simulink model "furuta_block_model_fixed"  (R2026b)
settings: Solver=FixedStepDiscrete  StopTime=5  FixedStep=.005  EnableMultiTasking=on
InitFcn:
  | validate_furuta_fixed_test('furuta_block_model_fixed');
model workspace (MAT data in the model file):
  calibration = [73.65 -1 4058.5 1]
  controlPeriod = 0.01
  drive = [-1 1.5 1.5 inf]
  driveElectrical : object (value not decoded)
  failureReplayEnabled = 0
  failureReplaySlowdown = 10
  failureReplaySource = 'C:\Capstone1\matlab_furuta\results\ppo_rmd_candidate_tpa79dc374_f9fe_4d66_a12a_2e210f4a8415\ppo_start_-20_+20_armrate_20_current_1.5_time_10_armlimit_Inf.mat'
  failureReplayStartDeg = 20
  failureReplayState = [0 0.1 0.2 0.3 0.4 0.5 0.6 0.7 0.8 0.9 1 1.1 ... (205 elements, 41x5)]
  furutaPPOAgent : rl.agent.rlPPOAgent (value not decoded)
  furutaSACAgent : rl.agent.rlSACAgent (value not decoded)
  furutaToolboxMpc : object (value not decoded)
  initialState = [0; 3.05432619099; 0; 0]
  integrationStep = 0.002
  limits = [inf 3.3 15 20]
  lqrGain = [-1.90684760658 -25.0276005412 -1.03983138576 -2.50199272238]
  maxTorque = 3.15
  milVelocityLimits = [15 25]
  pidGains = [25.0276005412 5.00398544475 1.90684760658 2.07966277151 0.001]
  plantCoefficients = [0.05 0.00016078 0.00016134 0.00013805 0.016934 0.0001 1e-05 0.63]
  rlRewardLevel = 2
  rmd : object (value not decoded)
  rmdCommandDelaySamples = 1
  scenarioStimulus = [0  0  0  0; 20  0  0  0]
  swingLqrThresholds = [0.226892802759 0.2 0.523598775598]
  usePolicyCallback = 0
  useRmd = 1
  velocityFilterTau = 0.03
values from neighbouring files (symbols this model uses):
  C = [B A*B A^2*B A^3*B]    [build_furuta_rmd.m]
  N = 20    [build_furuta_rl.m]    (also in design_classical.m)
  s = load(matFile,'ds')    [analyze_pi_current_run.m]    (also in analyze_pi_speed_run.m; build_furuta_rl.m = sin(x(2));"; build_furuta_simulink.m = s(1); design_classical.m = furuta_scenarios)
  source = [step '/1']    [add_furuta_plant_blocks.m]    (also in build_furuta_pi.m = get_param(line,'SrcPortHandle'); build_furuta_pi_hardware.m = 'Drive interlocks/3'; compare_furuta_actuators.m = get_param([harness '/Requested torque'],'PortHandles'))
  Z = expm([A B; zeros(1,5)]*p.Ts)    [furuta_linearize.m]
symbols that are objects in the model workspace (value not decoded): driveElectrical, rmd
undefined symbols (not defined in the file or in its folder): lmpcF, lmpcH, poleGain, sgn, X, Y
libraries: sm_lib x36, raspberrypiCommlib x9, nesl_utility x8, fl_lib x7, rllib x2, mpclib x1, slpidlib x1, ee_lib x1
(part 2 of 4)

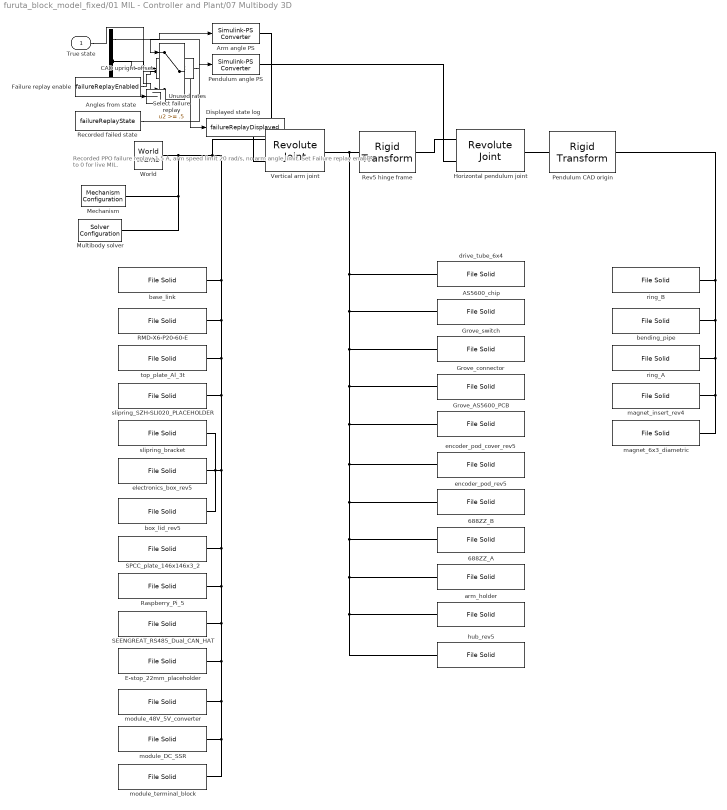
== system furuta_block_model_fixed/01 MIL - Controller and Plant/07 Multibody 3D ==
  note: Recorded PPO failure replay: 1.5 A, arm speed limit 20 rad/s, no arm angle limit. Set Failure replay enable to 0 for live MIL.
  True state : Inport
  688ZZ_A : sm_lib/Body Elements/File Solid  ExtGeomFileName=C:/Capstone1/models/rev5/source/meshes/688ZZ_A.stl  UnitType=Custom  ExtGeomFileUnits=mm  StepReaderType=HEX  ExportConvexHullGeometry=off  InertiaType=Custom  BasedOnType=DensityFromFile  Density=1000  DensityUnits=kg/m^3  Mass=0.005918760559363255  MassUnits=kg  CenterOfMass=[0.016 -2.788462968231947e-13 0.018]  CenterOfMassUnits=m  MomentsOfInertia=[2.367504233937143e-07 1.307059618430119e-07 1.307059638813835e-07]  MomentsOfInertiaUnits=kg*m^2  ProductsOfInertia=[7.843725669008149e-23 0 2.614575223002716e-23]  ProductsOfInertiaUnits=kg*m^2  GraphicType=FromGeometry  MarkerShape=Sphere  MarkerSize=10  GraphicVisPropType=SimpleVisualProperties  GraphicDiffuseColor=[.20 .50 .78]  GraphicOpacity=1  GraphicSpecularColor=[0.5 0.5 0.5 1.0]  GraphicAmbientColor=[0.15 0.15 0.15 1.0]  GraphicEmissiveColor=[0.0 0.0 0.0 1.0]  GraphicShininess=75  DoExposeReferenceFrame=on  SerializedFrames=<Frames/>
  688ZZ_B : sm_lib/Body Elements/File Solid  ExtGeomFileName=C:/Capstone1/models/rev5/source/meshes/688ZZ_B.stl  UnitType=Custom  ExtGeomFileUnits=mm  StepReaderType=HEX  ExportConvexHullGeometry=off  InertiaType=Custom  BasedOnType=DensityFromFile  Density=1000  DensityUnits=kg/m^3  Mass=0.005918760559363255  MassUnits=kg  CenterOfMass=[-0.016 -2.788462968231947e-13 0.018]  CenterOfMassUnits=m  MomentsOfInertia=[2.367504233937143e-07 1.307059618430119e-07 1.307059638813835e-07]  MomentsOfInertiaUnits=kg*m^2  ProductsOfInertia=[7.843725669008149e-23 4.235164736271502e-22 -1.13298259663451e-22]  ProductsOfInertiaUnits=kg*m^2  GraphicType=FromGeometry  MarkerShape=Sphere  MarkerSize=10  GraphicVisPropType=SimpleVisualProperties  GraphicDiffuseColor=[.20 .50 .78]  GraphicOpacity=1  GraphicSpecularColor=[0.5 0.5 0.5 1.0]  GraphicAmbientColor=[0.15 0.15 0.15 1.0]  GraphicEmissiveColor=[0.0 0.0 0.0 1.0]  GraphicShininess=75  DoExposeReferenceFrame=on  SerializedFrames=<Frames/>
  AS5600_chip : sm_lib/Body Elements/File Solid  ExtGeomFileName=C:/Capstone1/models/rev5/source/meshes/AS5600_chip.stl  UnitType=Custom  ExtGeomFileUnits=mm  StepReaderType=HEX  ExportConvexHullGeometry=off  InertiaType=Custom  BasedOnType=DensityFromFile  Density=1000  DensityUnits=kg/m^3  Mass=0.0002354999999999998  MassUnits=kg  CenterOfMass=[-0.02765 0 0.018]  CenterOfMassUnits=m  MomentsOfInertia=[8.04625000000029e-10 3.581562500000463e-10 5.347812500000514e-10]  MomentsOfInertiaUnits=kg*m^2  ProductsOfInertia=[-3.404394821604484e-25 2.646977960169689e-23 1.021318446481345e-24]  ProductsOfInertiaUnits=kg*m^2  GraphicType=FromGeometry  MarkerShape=Sphere  MarkerSize=10  GraphicVisPropType=SimpleVisualProperties  GraphicDiffuseColor=[.20 .50 .78]  GraphicOpacity=1  GraphicSpecularColor=[0.5 0.5 0.5 1.0]  GraphicAmbientColor=[0.15 0.15 0.15 1.0]  GraphicEmissiveColor=[0.0 0.0 0.0 1.0]  GraphicShininess=75  DoExposeReferenceFrame=on  SerializedFrames=<Frames/>
  Angles from state : Demux  Outputs=[1 1 2]
  Arm angle PS : nesl_utility/Simulink-PS Converter  PhysicalDomain=network_engine_domain  SubClassName=ps_input  LeftPortType=input  RightPortType=output  PseudoPeriodic=off  Frequencies=[]  NoiseDistribution=none  NoiseParameters=[]  Unit=rad  AffineConversion=off  FilteringAndDerivatives=filter  SimscapeFilterOrder=2  InputFilterTimeConstant=.003  UdotUserProvided=0
  CAD upright offset : Bias  Bias=-pi/2  SaturateOnIntegerOverflow=off
  Displayed state log : ToWorkspace  VariableName=failureReplayDisplayed  SaveFormat=Timeseries  SampleTime=-1
  E-stop_22mm_placeholder : sm_lib/Body Elements/File Solid  ExtGeomFileName=C:/Capstone1/models/rev5/source/meshes/E-stop_22mm_placeholder.stl  UnitType=Custom  ExtGeomFileUnits=mm  StepReaderType=HEX  ExportConvexHullGeometry=off  InertiaType=Custom  BasedOnType=DensityFromFile  Density=1000  DensityUnits=kg/m^3  Mass=0.1193616712804906  MassUnits=kg  CenterOfMass=[0.04499999999999998 -0.0525 -0.1708]  CenterOfMassUnits=m  MomentsOfInertia=[1.952558006030128e-05 7.221381112470972e-06 1.95255800603003e-05]  MomentsOfInertiaUnits=kg*m^2  ProductsOfInertia=[-8.673617379884035e-19 8.673617379884035e-19 0]  ProductsOfInertiaUnits=kg*m^2  GraphicType=FromGeometry  MarkerShape=Sphere  MarkerSize=10  GraphicVisPropType=SimpleVisualProperties  GraphicDiffuseColor=[.42 .43 .46]  GraphicOpacity=1  GraphicSpecularColor=[0.5 0.5 0.5 1.0]  GraphicAmbientColor=[0.15 0.15 0.15 1.0]  GraphicEmissiveColor=[0.0 0.0 0.0 1.0]  GraphicShininess=75  DoExposeReferenceFrame=on  SerializedFrames=<Frames/>
  Failure replay enable : Constant  Value=failureReplayEnabled
  Grove_AS5600_PCB : sm_lib/Body Elements/File Solid  ExtGeomFileName=C:/Capstone1/models/rev5/source/meshes/Grove_AS5600_PCB.stl  UnitType=Custom  ExtGeomFileUnits=mm  StepReaderType=HEX  ExportConvexHullGeometry=off  InertiaType=Custom  BasedOnType=DensityFromFile  Density=1000  DensityUnits=kg/m^3  Mass=0.0023511221076278556  MassUnits=kg  CenterOfMass=[-0.0292 -0.009998882871009487 0.018]  CenterOfMassUnits=m  MomentsOfInertia=[3.903658018417303e-07 7.840966792904181e-08 3.129592793452765e-07]  MomentsOfInertiaUnits=kg*m^2  ProductsOfInertia=[1.058791184067875e-22 2.117582368135751e-22 0]  ProductsOfInertiaUnits=kg*m^2  GraphicType=FromGeometry  MarkerShape=Sphere  MarkerSize=10  GraphicVisPropType=SimpleVisualProperties  GraphicDiffuseColor=[.20 .50 .78]  GraphicOpacity=1  GraphicSpecularColor=[0.5 0.5 0.5 1.0]  GraphicAmbientColor=[0.15 0.15 0.15 1.0]  GraphicEmissiveColor=[0.0 0.0 0.0 1.0]  GraphicShininess=75  DoExposeReferenceFrame=on  SerializedFrames=<Frames/>
  Grove_connector : sm_lib/Body Elements/File Solid  ExtGeomFileName=C:/Capstone1/models/rev5/source/meshes/Grove_connector.stl  UnitType=Custom  ExtGeomFileUnits=mm  StepReaderType=HEX  ExportConvexHullGeometry=off  InertiaType=Custom  BasedOnType=DensityFromFile  Density=1000  DensityUnits=kg/m^3  Mass=0.0005172800000000002  MassUnits=kg  CenterOfMass=[-0.0325 -0.02 0.018]  CenterOfMassUnits=m  MomentsOfInertia=[9.174822933333419e-09 7.493662933333236e-09 3.836493333333296e-09]  MomentsOfInertiaUnits=kg*m^2  ProductsOfInertia=[2.646977960169689e-23 0 0]  ProductsOfInertiaUnits=kg*m^2  GraphicType=FromGeometry  MarkerShape=Sphere  MarkerSize=10  GraphicVisPropType=SimpleVisualProperties  GraphicDiffuseColor=[.20 .50 .78]  GraphicOpacity=1  GraphicSpecularColor=[0.5 0.5 0.5 1.0]  GraphicAmbientColor=[0.15 0.15 0.15 1.0]  GraphicEmissiveColor=[0.0 0.0 0.0 1.0]  GraphicShininess=75  DoExposeReferenceFrame=on  SerializedFrames=<Frames/>
  Grove_switch : sm_lib/Body Elements/File Solid  ExtGeomFileName=C:/Capstone1/models/rev5/source/meshes/Grove_switch.stl  UnitType=Custom  ExtGeomFileUnits=mm  StepReaderType=HEX  ExportConvexHullGeometry=off  InertiaType=Custom  BasedOnType=DensityFromFile  Density=1000  DensityUnits=kg/m^3  Mass=6.268416000000009e-05  MassUnits=kg  CenterOfMass=[-0.0316 -0.0139 0.01292]  CenterOfMassUnits=m  MomentsOfInertia=[2.684971520000019e-10 2.810339839999896e-10 9.444413439999819e-11]  MomentsOfInertiaUnits=kg*m^2  ProductsOfInertia=[0 -3.308722450212111e-24 -3.308722450212111e-24]  ProductsOfInertiaUnits=kg*m^2  GraphicType=FromGeometry  MarkerShape=Sphere  MarkerSize=10  GraphicVisPropType=SimpleVisualProperties  GraphicDiffuseColor=[.20 .50 .78]  GraphicOpacity=1  GraphicSpecularColor=[0.5 0.5 0.5 1.0]  GraphicAmbientColor=[0.15 0.15 0.15 1.0]  GraphicEmissiveColor=[0.0 0.0 0.0 1.0]  GraphicShininess=75  DoExposeReferenceFrame=on  SerializedFrames=<Frames/>
  Horizontal pendulum joint : sm_lib/Joints/Revolute Joint  JointMode=Normal  CompositeWrenchDir=FollowerOnBase  CompositeWrenchFrame=BaseFrame  SenseConstraintForce=off  SenseConstraintTorque=off  SenseTotalForce=off  SenseTotalTorque=off  PositionTargetSpecify=off  PositionTargetPriority=High  PositionTargetValue=0  PositionTargetValueUnits=deg  VelocityTargetSpecify=off  VelocityTargetPriority=High  VelocityTargetValue=0  VelocityTargetValueUnits=deg/s  EquilibriumPosition=0  EquilibriumPositionUnits=deg  SpringStiffness=0  SpringStiffnessUnits=N*m/deg  DampingCoefficient=0  DampingCoefficientUnits=N*m/(deg/s)  LowerLimitSpecify=off  LowerLimitBound=-90  LowerLimitBoundUnits=deg  LowerLimitStiffness=1e4  LowerLimitStiffnessUnits=N*m/deg  LowerLimitDamping=10  LowerLimitDampingUnits=N*m/(deg/s)  LowerLimitTransitionRegionWidth=0.1  LowerLimitTransitionRegionWidthUnits=deg  UpperLimitSpecify=off  UpperLimitBound=90  UpperLimitBoundUnits=deg  UpperLimitStiffness=1e4  UpperLimitStiffnessUnits=N*m/deg  UpperLimitDamping=10  UpperLimitDampingUnits=N*m/(deg/s)  UpperLimitTransitionRegionWidth=0.1  UpperLimitTransitionRegionWidthUnits=deg  TorqueActuationMode=ComputedTorque  MotionActuationMode=InputMotion  SensePosition=off  SenseVelocity=off  SenseAcceleration=off  SenseTorqueForce=off  SenseLowerLimitTorqueForce=off  SenseUpperLimitTorqueForce=off
  Mechanism : sm_lib/Utilities/Mechanism Configuration  UniformGravity=Constant  GravityVector=[0 0 -9.80665]  GravityVectorUnits=m/s^2  LinearizationDelta=0.001  JointModeTransitionNonlinearIterations=2
  Multibody solver : nesl_utility/Solver Configuration  PhysicalDomain=network_engine_domain  SubClassName=solver  LeftPortType=input  RightPortType=generic  Tones=[]  Harmonics=[]  SimulateNoise=off  Profile=off  UseLocalSampling=off  EnableSwitchedLinearOptims=on  FrequencyDomain=off  UseCCode=off  RelTol=0.001  AbsTol=0.001  MinStep=1e-09  ToWorkspace=off  RevertToSquareIcSolve=off  NumHomotopyIterations=100  PhasorMode=off  PhasorModeNumHarmonics=1  ConsistencySolver=NEWTON_XTOL_AFTER_FTOL  CanonicalOrdering=CANONICAL  OptimizeIntermediates=OPTIMIZED  MulticoreSolverChoice=BACKWARD_EULER  IndexReductionMethod=DerivativeReplacement  DoDC=off  ResidualTolerance=1e-09  ConsistencyTolSource=GLOBAL  ConsistencyAbsTol=0.001  ConsistencyRelTol=0.001  ConsistencyTolFactor=0.001  UseLocalSolver=off  LocalSolverChoice=NE_BACKWARD_EULER_ADVANCER  ResolveIndetEquations=on  FunctionEvalNumThread=1  LocalSolverSampleTime=0.001  DoFixedCost=off  MaxNonlinIter=3  MaxModeIter=2  ComputeImpulses=off  ImpulseIterations=2  LinearAlgebra=auto  LinearAlgebraNumThread=0  EquationFormulation=NE_TIME_EF  DelaysMemoryBudget=1024  AutomaticFiltering=on  FilteringTimeConstant=0.001  PartitionStorageMethod=AS_NEEDED  PartitionMemoryBudget=1024  PartitionMethod=BALANCED  MultibodyUseLocalSolver=off  MultibodyLocalSolverChoice=ODE1  MultibodyLocalSolverSampleTime=0.001
  Pendulum CAD origin : sm_lib/Frames and Transforms/Rigid Transform  RotationMethod=RotationMatrix  FollAlignAxisA=+X  BaseAlignAxisA=+Y  FollAlignAxisB=+Y  BaseAlignAxisB=+Z  RotationStandardAxis=+Z  RotationAngle=0  RotationAngleUnits=deg  RotationArbitraryAxis=[0 0 1]  RotationSequenceAxes=FollowerAxes  RotationSequence=XYX  RotationSequenceAngles=[0 0 0]  RotationSequenceAnglesUnits=deg  RotationMatrix=[0 0 -1;0 1 0;1 0 0]  Quaternion=[1 0 0 0]  TranslationMethod=Cartesian  TranslationCartesianOffset=[0.018 0 0.0185]  TranslationCartesianOffsetUnits=m  TranslationStandardAxis=+Z  TranslationStandardOffset=0  TranslationStandardOffsetUnits=m  TranslationROffset=0  TranslationROffsetUnits=m  TranslationThetaOffset=0  TranslationThetaOffsetUnits=deg  TranslationZOffset=0  TranslationZOffsetUnits=m
  Pendulum angle PS : nesl_utility/Simulink-PS Converter  PhysicalDomain=network_engine_domain  SubClassName=ps_input  LeftPortType=input  RightPortType=output  PseudoPeriodic=off  Frequencies=[]  NoiseDistribution=none  NoiseParameters=[]  Unit=rad  AffineConversion=off  FilteringAndDerivatives=filter  SimscapeFilterOrder=2  InputFilterTimeConstant=.003  UdotUserProvided=0
  RMD-X6-P20-60-E : sm_lib/Body Elements/File Solid  ExtGeomFileName=C:/Capstone1/models/rev5/source/meshes/RMD-X6-P20-60-E.stl  UnitType=Custom  ExtGeomFileUnits=mm  StepReaderType=HEX  ExportConvexHullGeometry=off  InertiaType=Custom  BasedOnType=DensityFromFile  Density=1000  DensityUnits=kg/m^3  Mass=0.5295460172821769  MassUnits=kg  CenterOfMass=[-8.898918041415573e-05 -0.0001349554467787079 -0.02861574603154959]  CenterOfMassUnits=m  MomentsOfInertia=[0.0005329118585045489 0.0005318244984692392 0.0005420384995759367]  MomentsOfInertiaUnits=kg*m^2  ProductsOfInertia=[-2.743134480207274e-06 -1.937494531495924e-06 7.067599187778668e-07]  ProductsOfInertiaUnits=kg*m^2  GraphicType=FromGeometry  MarkerShape=Sphere  MarkerSize=10  GraphicVisPropType=SimpleVisualProperties  GraphicDiffuseColor=[.42 .43 .46]  GraphicOpacity=1  GraphicSpecularColor=[0.5 0.5 0.5 1.0]  GraphicAmbientColor=[0.15 0.15 0.15 1.0]  GraphicEmissiveColor=[0.0 0.0 0.0 1.0]  GraphicShininess=75  DoExposeReferenceFrame=on  SerializedFrames=<Frames/>
  Raspberry_Pi_5 : sm_lib/Body Elements/File Solid  ExtGeomFileName=C:/Capstone1/models/rev5/source/meshes/Raspberry_Pi_5.stl  UnitType=Custom  ExtGeomFileUnits=mm  StepReaderType=HEX  ExportConvexHullGeometry=off  InertiaType=Custom  BasedOnType=DensityFromFile  Density=1000  DensityUnits=kg/m^3  Mass=0.15621931750000087  MassUnits=kg  CenterOfMass=[-0.03256410689654306 -0.04863618844705284 -0.1777024256867273]  CenterOfMassUnits=m  MomentsOfInertia=[0.0001079953099151851 4.200239752131033e-05 0.0001411220451968511]  MomentsOfInertiaUnits=kg*m^2  ProductsOfInertia=[1.076566474419332e-05 -2.39989746857682e-07 1.077911171535483e-05]  ProductsOfInertiaUnits=kg*m^2  GraphicType=FromGeometry  MarkerShape=Sphere  MarkerSize=10  GraphicVisPropType=SimpleVisualProperties  GraphicDiffuseColor=[.42 .43 .46]  GraphicOpacity=1  GraphicSpecularColor=[0.5 0.5 0.5 1.0]  GraphicAmbientColor=[0.15 0.15 0.15 1.0]  GraphicEmissiveColor=[0.0 0.0 0.0 1.0]  GraphicShininess=75  DoExposeReferenceFrame=on  SerializedFrames=<Frames/>
  Recorded failed state : FromWorkspace  VariableName=failureReplayState  OutputAfterFinalValue=Holding final value
  Rev5 hinge frame : sm_lib/Frames and Transforms/Rigid Transform  RotationMethod=RotationMatrix  FollAlignAxisA=+X  BaseAlignAxisA=+Y  FollAlignAxisB=+Y  BaseAlignAxisB=+Z  RotationStandardAxis=+Z  RotationAngle=0  RotationAngleUnits=deg  RotationArbitraryAxis=[0 0 1]  RotationSequenceAxes=FollowerAxes  RotationSequence=XYX  RotationSequenceAngles=[0 0 0]  RotationSequenceAnglesUnits=deg  RotationMatrix=[0 0 1;0 1 0;-1 0 0]  Quaternion=[1 0 0 0]  TranslationMethod=Cartesian  TranslationCartesianOffset=[-0.0185 0 0.018]  TranslationCartesianOffsetUnits=m  TranslationStandardAxis=+Z  TranslationStandardOffset=0  TranslationStandardOffsetUnits=m  TranslationROffset=0  TranslationROffsetUnits=m  TranslationThetaOffset=0  TranslationThetaOffsetUnits=deg  TranslationZOffset=0  TranslationZOffsetUnits=m
  SEENGREAT_RS485_Dual_CAN_HAT : sm_lib/Body Elements/File Solid  ExtGeomFileName=C:/Capstone1/models/rev5/source/meshes/SEENGREAT_RS485_Dual_CAN_HAT.stl  UnitType=Custom  ExtGeomFileUnits=mm  StepReaderType=HEX  ExportConvexHullGeometry=off  InertiaType=Custom  BasedOnType=DensityFromFile  Density=1000  DensityUnits=kg/m^3  Mass=0.12528993684249518  MassUnits=kg  CenterOfMass=[-0.0485018721946214 -0.017999998175319 -0.1686245785232124]  CenterOfMassUnits=m  MomentsOfInertia=[3.479562574944207e-05 4.034313002730444e-05 7.275959915954754e-05]  MomentsOfInertiaUnits=kg*m^2  ProductsOfInertia=[-1.084202172485504e-19 2.723311433297168e-06 4.065758146820642e-20]  ProductsOfInertiaUnits=kg*m^2  GraphicType=FromGeometry  MarkerShape=Sphere  MarkerSize=10  GraphicVisPropType=SimpleVisualProperties  GraphicDiffuseColor=[.42 .43 .46]  GraphicOpacity=1  GraphicSpecularColor=[0.5 0.5 0.5 1.0]  GraphicAmbientColor=[0.15 0.15 0.15 1.0]  GraphicEmissiveColor=[0.0 0.0 0.0 1.0]  GraphicShininess=75  DoExposeReferenceFrame=on  SerializedFrames=<Frames/>
  SPCC_plate_146x146x3_2 : sm_lib/Body Elements/File Solid  ExtGeomFileName=C:/Capstone1/models/rev5/source/meshes/SPCC_plate_146x146x3_2.stl  UnitType=Custom  ExtGeomFileUnits=mm  StepReaderType=HEX  ExportConvexHullGeometry=off  InertiaType=Custom  BasedOnType=DensityFromFile  Density=1000  DensityUnits=kg/m^3  Mass=0.5340065618922325  MassUnits=kg  CenterOfMass=[-2.455775156158338e-05 -5.018323145254561e-05 -0.1934]  CenterOfMassUnits=m  MomentsOfInertia=[0.0009454567177696153 0.0009456802224071248 0.001890225568977773]  MomentsOfInertiaUnits=kg*m^2  ProductsOfInertia=[-2.117582368135751e-19 -2.757092243312748e-19 -9.230236699785122e-07]  ProductsOfInertiaUnits=kg*m^2  GraphicType=FromGeometry  MarkerShape=Sphere  MarkerSize=10  GraphicVisPropType=SimpleVisualProperties  GraphicDiffuseColor=[.42 .43 .46]  GraphicOpacity=1  GraphicSpecularColor=[0.5 0.5 0.5 1.0]  GraphicAmbientColor=[0.15 0.15 0.15 1.0]  GraphicEmissiveColor=[0.0 0.0 0.0 1.0]  GraphicShininess=75  DoExposeReferenceFrame=on  SerializedFrames=<Frames/>
  Select failure replay : Switch  Threshold=.5  SaturateOnIntegerOverflow=off  InputSameDT=off
  Unused rates : Terminator
  Vertical arm joint : sm_lib/Joints/Revolute Joint  JointMode=Normal  CompositeWrenchDir=FollowerOnBase  CompositeWrenchFrame=BaseFrame  SenseConstraintForce=off  SenseConstraintTorque=off  SenseTotalForce=off  SenseTotalTorque=off  PositionTargetSpecify=off  PositionTargetPriority=High  PositionTargetValue=0  PositionTargetValueUnits=deg  VelocityTargetSpecify=off  VelocityTargetPriority=High  VelocityTargetValue=0  VelocityTargetValueUnits=deg/s  EquilibriumPosition=0  EquilibriumPositionUnits=deg  SpringStiffness=0  SpringStiffnessUnits=N*m/deg  DampingCoefficient=0  DampingCoefficientUnits=N*m/(deg/s)  LowerLimitSpecify=off  LowerLimitBound=-90  LowerLimitBoundUnits=deg  LowerLimitStiffness=1e4  LowerLimitStiffnessUnits=N*m/deg  LowerLimitDamping=10  LowerLimitDampingUnits=N*m/(deg/s)  LowerLimitTransitionRegionWidth=0.1  LowerLimitTransitionRegionWidthUnits=deg  UpperLimitSpecify=off  UpperLimitBound=90  UpperLimitBoundUnits=deg  UpperLimitStiffness=1e4  UpperLimitStiffnessUnits=N*m/deg  UpperLimitDamping=10  UpperLimitDampingUnits=N*m/(deg/s)  UpperLimitTransitionRegionWidth=0.1  UpperLimitTransitionRegionWidthUnits=deg  TorqueActuationMode=ComputedTorque  MotionActuationMode=InputMotion  SensePosition=off  SenseVelocity=off  SenseAcceleration=off  SenseTorqueForce=off  SenseLowerLimitTorqueForce=off  SenseUpperLimitTorqueForce=off
  World : sm_lib/Frames and Transforms/World Frame
  arm_holder : sm_lib/Body Elements/File Solid  ExtGeomFileName=C:/Capstone1/models/rev5/source/meshes/arm_holder.stl  UnitType=Custom  ExtGeomFileUnits=mm  StepReaderType=HEX  ExportConvexHullGeometry=off  InertiaType=Custom  BasedOnType=DensityFromFile  Density=1000  DensityUnits=kg/m^3  Mass=0.017663069712980626  MassUnits=kg  CenterOfMass=[-2.842448076868302e-12 -5.768473624794685e-07 0.01590591778152516]  CenterOfMassUnits=m  MomentsOfInertia=[2.503616629279688e-06 2.567289522841808e-06 3.706027090878154e-06]  MomentsOfInertiaUnits=kg*m^2  ProductsOfInertia=[6.016343314434523e-12 -2.965155067037797e-16 4.291361716321984e-21]  ProductsOfInertiaUnits=kg*m^2  GraphicType=FromGeometry  MarkerShape=Sphere  MarkerSize=10  GraphicVisPropType=SimpleVisualProperties  GraphicDiffuseColor=[.20 .50 .78]  GraphicOpacity=1  GraphicSpecularColor=[0.5 0.5 0.5 1.0]  GraphicAmbientColor=[0.15 0.15 0.15 1.0]  GraphicEmissiveColor=[0.0 0.0 0.0 1.0]  GraphicShininess=75  DoExposeReferenceFrame=on  SerializedFrames=<Frames/>
  base_link : sm_lib/Body Elements/File Solid  ExtGeomFileName=C:/Capstone1/models/rev5/source/meshes/base_link.stl  UnitType=Custom  ExtGeomFileUnits=mm  StepReaderType=HEX  ExportConvexHullGeometry=off  InertiaType=Custom  BasedOnType=DensityFromFile  Density=1000  DensityUnits=kg/m^3  Mass=1.4818316319511198  MassUnits=kg  CenterOfMass=[6.478814537983507e-05 -2.78394022838701e-06 -0.08720518232484926]  CenterOfMassUnits=m  MomentsOfInertia=[0.005497507249541402 0.00550186713597068 0.003671506569899864]  MomentsOfInertiaUnits=kg*m^2  ProductsOfInertia=[-6.515884611751008e-08 3.004462826416078e-06 -2.672725224527317e-10]  ProductsOfInertiaUnits=kg*m^2  GraphicType=FromGeometry  MarkerShape=Sphere  MarkerSize=10  GraphicVisPropType=SimpleVisualProperties  GraphicDiffuseColor=[.42 .43 .46]  GraphicOpacity=1  GraphicSpecularColor=[0.5 0.5 0.5 1.0]  GraphicAmbientColor=[0.15 0.15 0.15 1.0]  GraphicEmissiveColor=[0.0 0.0 0.0 1.0]  GraphicShininess=75  DoExposeReferenceFrame=on  SerializedFrames=<Frames/>
  bending_pipe : sm_lib/Body Elements/File Solid  ExtGeomFileName=C:/Capstone1/models/rev5/source/meshes/bending_pipe.stl  UnitType=Custom  ExtGeomFileUnits=mm  StepReaderType=HEX  ExportConvexHullGeometry=off  InertiaType=Custom  BasedOnType=DensityFromFile  Density=1000  DensityUnits=kg/m^3  Mass=0.0404810331676941  MassUnits=kg  CenterOfMass=[0.05804143296811888 -0.0418429445646091 0.01799792411906267]  CenterOfMassUnits=m  MomentsOfInertia=[8.739271874299467e-05 4.082210915887574e-05 0.000127709095047693]  MomentsOfInertiaUnits=kg*m^2  ProductsOfInertia=[3.448904757875307e-09 -6.473777685567206e-09 3.715262539327471e-05]  ProductsOfInertiaUnits=kg*m^2  GraphicType=FromGeometry  MarkerShape=Sphere  MarkerSize=10  GraphicVisPropType=SimpleVisualProperties  GraphicDiffuseColor=[.89 .48 .19]  GraphicOpacity=1  GraphicSpecularColor=[0.5 0.5 0.5 1.0]  GraphicAmbientColor=[0.15 0.15 0.15 1.0]  GraphicEmissiveColor=[0.0 0.0 0.0 1.0]  GraphicShininess=75  DoExposeReferenceFrame=on  SerializedFrames=<Frames/>
  box_lid_rev5 : sm_lib/Body Elements/File Solid  ExtGeomFileName=C:/Capstone1/models/rev5/source/meshes/box_lid_rev5.stl  UnitType=Custom  ExtGeomFileUnits=mm  StepReaderType=HEX  ExportConvexHullGeometry=off  InertiaType=Custom  BasedOnType=DensityFromFile  Density=1000  DensityUnits=kg/m^3  Mass=0.3820749661262098  MassUnits=kg  CenterOfMass=[-9.02544061665338e-05 -0.0001822143245718956 -0.1516519532976607]  CenterOfMassUnits=m  MomentsOfInertia=[0.000956654363030076 0.0009570108829092244 0.001912765627368311]  MomentsOfInertiaUnits=kg*m^2  ProductsOfInertia=[-4.757483789999227e-08 -2.446272057208077e-08 -2.414109308533263e-06]  ProductsOfInertiaUnits=kg*m^2  GraphicType=FromGeometry  MarkerShape=Sphere  MarkerSize=10  GraphicVisPropType=SimpleVisualProperties  GraphicDiffuseColor=[.42 .43 .46]  GraphicOpacity=1  GraphicSpecularColor=[0.5 0.5 0.5 1.0]  GraphicAmbientColor=[0.15 0.15 0.15 1.0]  GraphicEmissiveColor=[0.0 0.0 0.0 1.0]  GraphicShininess=75  DoExposeReferenceFrame=on  SerializedFrames=<Frames/>
  drive_tube_6x4 : sm_lib/Body Elements/File Solid  ExtGeomFileName=C:/Capstone1/models/rev5/source/meshes/drive_tube_6x4.stl  UnitType=Custom  ExtGeomFileUnits=mm  StepReaderType=HEX  ExportConvexHullGeometry=off  InertiaType=Custom  BasedOnType=DensityFromFile  Density=1000  DensityUnits=kg/m^3  Mass=0.009556332153138622  MassUnits=kg  CenterOfMass=[-1.67308576082546e-13 0 -0.0337500000000003]  CenterOfMassUnits=m  MomentsOfInertia=[4.814201412149952e-06 4.814201413137291e-06 6.211615948906929e-08]  MomentsOfInertiaUnits=kg*m^2  ProductsOfInertia=[-5.229150445984487e-22 -3.09783042967688e-17 3.268219028740304e-23]  ProductsOfInertiaUnits=kg*m^2  GraphicType=FromGeometry  MarkerShape=Sphere  MarkerSize=10  GraphicVisPropType=SimpleVisualProperties  GraphicDiffuseColor=[.20 .50 .78]  GraphicOpacity=1  GraphicSpecularColor=[0.5 0.5 0.5 1.0]  GraphicAmbientColor=[0.15 0.15 0.15 1.0]  GraphicEmissiveColor=[0.0 0.0 0.0 1.0]  GraphicShininess=75  DoExposeReferenceFrame=on  SerializedFrames=<Frames/>
  electronics_box_rev5 : sm_lib/Body Elements/File Solid  ExtGeomFileName=C:/Capstone1/models/rev5/source/meshes/electronics_box_rev5.stl  UnitType=Custom  ExtGeomFileUnits=mm  StepReaderType=HEX  ExportConvexHullGeometry=off  InertiaType=Custom  BasedOnType=DensityFromFile  Density=1000  DensityUnits=kg/m^3  Mass=0.8208148864821171  MassUnits=kg  CenterOfMass=[0.002742198181315165 0.004689009623718564 -0.1800114945579828]  CenterOfMassUnits=m  MomentsOfInertia=[0.00237449428694118 0.002458771924756679 0.004573095057647558]  MomentsOfInertiaUnits=kg*m^2  ProductsOfInertia=[-2.748739163888287e-05 -8.794224210412725e-06 0.0001000738159775882]  ProductsOfInertiaUnits=kg*m^2  GraphicType=FromGeometry  MarkerShape=Sphere  MarkerSize=10  GraphicVisPropType=SimpleVisualProperties  GraphicDiffuseColor=[.42 .43 .46]  GraphicOpacity=1  GraphicSpecularColor=[0.5 0.5 0.5 1.0]  GraphicAmbientColor=[0.15 0.15 0.15 1.0]  GraphicEmissiveColor=[0.0 0.0 0.0 1.0]  GraphicShininess=75  DoExposeReferenceFrame=on  SerializedFrames=<Frames/>
  encoder_pod_cover_rev5 : sm_lib/Body Elements/File Solid  ExtGeomFileName=C:/Capstone1/models/rev5/source/meshes/encoder_pod_cover_rev5.stl  UnitType=Custom  ExtGeomFileUnits=mm  StepReaderType=HEX  ExportConvexHullGeometry=off  InertiaType=Custom  BasedOnType=DensityFromFile  Density=1000  DensityUnits=kg/m^3  Mass=0.0029898563826147324  MassUnits=kg  CenterOfMass=[-0.03668117274392343 -0.005387765769535873 0.01799999999999999]  CenterOfMassUnits=m  MomentsOfInertia=[8.62392468753039e-07 1.94131783288769e-07 6.72673097439614e-07]  MomentsOfInertiaUnits=kg*m^2  ProductsOfInertia=[-2.117582368135751e-22 0 -2.269422618409756e-09]  ProductsOfInertiaUnits=kg*m^2  GraphicType=FromGeometry  MarkerShape=Sphere  MarkerSize=10  GraphicVisPropType=SimpleVisualProperties  GraphicDiffuseColor=[.20 .50 .78]  GraphicOpacity=1  GraphicSpecularColor=[0.5 0.5 0.5 1.0]  GraphicAmbientColor=[0.15 0.15 0.15 1.0]  GraphicEmissiveColor=[0.0 0.0 0.0 1.0]  GraphicShininess=75  DoExposeReferenceFrame=on  SerializedFrames=<Frames/>
  encoder_pod_rev5 : sm_lib/Body Elements/File Solid  ExtGeomFileName=C:/Capstone1/models/rev5/source/meshes/encoder_pod_rev5.stl  UnitType=Custom  ExtGeomFileUnits=mm  StepReaderType=HEX  ExportConvexHullGeometry=off  InertiaType=Custom  BasedOnType=DensityFromFile  Density=1000  DensityUnits=kg/m^3  Mass=0.021327607571930463  MassUnits=kg  CenterOfMass=[-0.02566834845138082 -0.004921423811282861 0.01894684101790099]  CenterOfMassUnits=m  MomentsOfInertia=[7.697431517849671e-06 1.995769022994516e-06 6.68909847511237e-06]  MomentsOfInertiaUnits=kg*m^2  ProductsOfInertia=[-6.620085789305091e-09 2.907995322212918e-09 2.834056722013257e-07]  ProductsOfInertiaUnits=kg*m^2  GraphicType=FromGeometry  MarkerShape=Sphere  MarkerSize=10  GraphicVisPropType=SimpleVisualProperties  GraphicDiffuseColor=[.20 .50 .78]  GraphicOpacity=1  GraphicSpecularColor=[0.5 0.5 0.5 1.0]  GraphicAmbientColor=[0.15 0.15 0.15 1.0]  GraphicEmissiveColor=[0.0 0.0 0.0 1.0]  GraphicShininess=75  DoExposeReferenceFrame=on  SerializedFrames=<Frames/>
  hub_rev5 : sm_lib/Body Elements/File Solid  ExtGeomFileName=C:/Capstone1/models/rev5/source/meshes/hub_rev5.stl  UnitType=Custom  ExtGeomFileUnits=mm  StepReaderType=HEX  ExportConvexHullGeometry=off  InertiaType=Custom  BasedOnType=DensityFromFile  Density=1000  DensityUnits=kg/m^3  Mass=0.019832305826006934  MassUnits=kg  CenterOfMass=[6.334948209511458e-06 4.442614994304577e-18 0.003846693050057123]  CenterOfMassUnits=m  MomentsOfInertia=[3.896570962818379e-06 3.431908871421857e-06 7.11816654744243e-06]  MomentsOfInertiaUnits=kg*m^2  ProductsOfInertia=[-1.863760745232609e-21 -1.12296899222146e-08 7.049142093917723e-21]  ProductsOfInertiaUnits=kg*m^2  GraphicType=FromGeometry  MarkerShape=Sphere  MarkerSize=10  GraphicVisPropType=SimpleVisualProperties  GraphicDiffuseColor=[.20 .50 .78]  GraphicOpacity=1  GraphicSpecularColor=[0.5 0.5 0.5 1.0]  GraphicAmbientColor=[0.15 0.15 0.15 1.0]  GraphicEmissiveColor=[0.0 0.0 0.0 1.0]  GraphicShininess=75  DoExposeReferenceFrame=on  SerializedFrames=<Frames/>
  magnet_6x3_diametric : sm_lib/Body Elements/File Solid  ExtGeomFileName=C:/Capstone1/models/rev5/source/meshes/magnet_6x3_diametric.stl  UnitType=Custom  ExtGeomFileUnits=mm  StepReaderType=HEX  ExportConvexHullGeometry=off  InertiaType=Custom  BasedOnType=DensityFromFile  Density=1000  DensityUnits=kg/m^3  Mass=0.0006658605629283288  MassUnits=kg  CenterOfMass=[-0.0234 6.274077672453813e-13 0.018]  CenterOfMassUnits=m  MomentsOfInertia=[2.996372339690661e-09 1.997581785528354e-09 1.997581398554788e-09]  MomentsOfInertiaUnits=kg*m^2  ProductsOfInertia=[3.676746408021645e-24 -5.293955920339377e-23 3.949097980847364e-25]  ProductsOfInertiaUnits=kg*m^2  GraphicType=FromGeometry  MarkerShape=Sphere  MarkerSize=10  GraphicVisPropType=SimpleVisualProperties  GraphicDiffuseColor=[.89 .48 .19]  GraphicOpacity=1  GraphicSpecularColor=[0.5 0.5 0.5 1.0]  GraphicAmbientColor=[0.15 0.15 0.15 1.0]  GraphicEmissiveColor=[0.0 0.0 0.0 1.0]  GraphicShininess=75  DoExposeReferenceFrame=on  SerializedFrames=<Frames/>
  magnet_insert_rev4 : sm_lib/Body Elements/File Solid  ExtGeomFileName=C:/Capstone1/models/rev5/source/meshes/magnet_insert_rev4.stl  UnitType=Custom  ExtGeomFileUnits=mm  StepReaderType=HEX  ExportConvexHullGeometry=off  InertiaType=Custom  BasedOnType=DensityFromFile  Density=1000  DensityUnits=kg/m^3  Mass=0.0003028220080455772  MassUnits=kg  CenterOfMass=[-0.02000375868372909 -8.958771672203236e-15 0.01811678890086537]  CenterOfMassUnits=m  MomentsOfInertia=[2.01880312561132e-09 3.053908917178372e-09 3.115381398386612e-09]  MomentsOfInertiaUnits=kg*m^2  ProductsOfInertia=[9.257947255001311e-21 8.668422003963615e-11 1.287064483427642e-21]  ProductsOfInertiaUnits=kg*m^2  GraphicType=FromGeometry  MarkerShape=Sphere  MarkerSize=10  GraphicVisPropType=SimpleVisualProperties  GraphicDiffuseColor=[.89 .48 .19]  GraphicOpacity=1  GraphicSpecularColor=[0.5 0.5 0.5 1.0]  GraphicAmbientColor=[0.15 0.15 0.15 1.0]  GraphicEmissiveColor=[0.0 0.0 0.0 1.0]  GraphicShininess=75  DoExposeReferenceFrame=on  SerializedFrames=<Frames/>
  module_48V_5V_converter : sm_lib/Body Elements/File Solid  ExtGeomFileName=C:/Capstone1/models/rev5/source/meshes/module_48V_5V_converter.stl  UnitType=Custom  ExtGeomFileUnits=mm  StepReaderType=HEX  ExportConvexHullGeometry=off  InertiaType=Custom  BasedOnType=DensityFromFile  Density=1000  DensityUnits=kg/m^3  Mass=0.2967299999999995  MassUnits=kg  CenterOfMass=[-0.033 0.036 -0.1808]  CenterOfMassUnits=m  MomentsOfInertia=[3.830289749999841e-05 9.703070999999772e-05 0.0001193101874999999]  MomentsOfInertiaUnits=kg*m^2  ProductsOfInertia=[-4.336808689942018e-19 2.168404344971009e-19 -1.084202172485504e-19]  ProductsOfInertiaUnits=kg*m^2  GraphicType=FromGeometry  MarkerShape=Sphere  MarkerSize=10  GraphicVisPropType=SimpleVisualProperties  GraphicDiffuseColor=[.42 .43 .46]  GraphicOpacity=1  GraphicSpecularColor=[0.5 0.5 0.5 1.0]  GraphicAmbientColor=[0.15 0.15 0.15 1.0]  GraphicEmissiveColor=[0.0 0.0 0.0 1.0]  GraphicShininess=75  DoExposeReferenceFrame=on  SerializedFrames=<Frames/>
  module_DC_SSR : sm_lib/Body Elements/File Solid  ExtGeomFileName=C:/Capstone1/models/rev5/source/meshes/module_DC_SSR.stl  UnitType=Custom  ExtGeomFileUnits=mm  StepReaderType=HEX  ExportConvexHullGeometry=off  InertiaType=Custom  BasedOnType=DensityFromFile  Density=1000  DensityUnits=kg/m^3  Mass=0.41966099999999984  MassUnits=kg  CenterOfMass=[0.034 0.0425 -0.1788]  CenterOfMassUnits=m  MomentsOfInertia=[8.774412074999578e-05 0.0001189039499999971 0.0001727954167500001]  MomentsOfInertiaUnits=kg*m^2  ProductsOfInertia=[-8.673617379884035e-19 0 0]  ProductsOfInertiaUnits=kg*m^2  GraphicType=FromGeometry  MarkerShape=Sphere  MarkerSize=10  GraphicVisPropType=SimpleVisualProperties  GraphicDiffuseColor=[.42 .43 .46]  GraphicOpacity=1  GraphicSpecularColor=[0.5 0.5 0.5 1.0]  GraphicAmbientColor=[0.15 0.15 0.15 1.0]  GraphicEmissiveColor=[0.0 0.0 0.0 1.0]  GraphicShininess=75  DoExposeReferenceFrame=on  SerializedFrames=<Frames/>
  module_terminal_block : sm_lib/Body Elements/File Solid  ExtGeomFileName=C:/Capstone1/models/rev5/source/meshes/module_terminal_block.stl  UnitType=Custom  ExtGeomFileUnits=mm  StepReaderType=HEX  ExportConvexHullGeometry=off  InertiaType=Custom  BasedOnType=DensityFromFile  Density=1000  DensityUnits=kg/m^3  Mass=0.08477999999999986  MassUnits=kg  CenterOfMass=[0.04 -0.0075 -0.1808]  CenterOfMassUnits=m  MomentsOfInertia=[3.878685000000427e-06 1.359306000000074e-05 1.289362499999998e-05]  MomentsOfInertiaUnits=kg*m^2  ProductsOfInertia=[1.355252715606881e-20 0 3.388131789017201e-21]  ProductsOfInertiaUnits=kg*m^2  GraphicType=FromGeometry  MarkerShape=Sphere  MarkerSize=10  GraphicVisPropType=SimpleVisualProperties  GraphicDiffuseColor=[.42 .43 .46]  GraphicOpacity=1  GraphicSpecularColor=[0.5 0.5 0.5 1.0]  GraphicAmbientColor=[0.15 0.15 0.15 1.0]  GraphicEmissiveColor=[0.0 0.0 0.0 1.0]  GraphicShininess=75  DoExposeReferenceFrame=on  SerializedFrames=<Frames/>
  ring_A : sm_lib/Body Elements/File Solid  ExtGeomFileName=C:/Capstone1/models/rev5/source/meshes/ring_A.stl  UnitType=Custom  ExtGeomFileUnits=mm  StepReaderType=HEX  ExportConvexHullGeometry=off  InertiaType=Custom  BasedOnType=DensityFromFile  Density=1000  DensityUnits=kg/m^3  Mass=0.0006658605629283556  MassUnits=kg  CenterOfMass=[0.02010000000000001 -2.454131698660125e-18 0.01800000000000001]  CenterOfMassUnits=m  MomentsOfInertia=[1.365014154003102e-08 7.324466192211724e-09 7.324466192211512e-09]  MomentsOfInertiaUnits=kg*m^2  ProductsOfInertia=[1.688579831515823e-23 1.058791184067875e-22 3.921862834488354e-24]  ProductsOfInertiaUnits=kg*m^2  GraphicType=FromGeometry  MarkerShape=Sphere  MarkerSize=10  GraphicVisPropType=SimpleVisualProperties  GraphicDiffuseColor=[.89 .48 .19]  GraphicOpacity=1  GraphicSpecularColor=[0.5 0.5 0.5 1.0]  GraphicAmbientColor=[0.15 0.15 0.15 1.0]  GraphicEmissiveColor=[0.0 0.0 0.0 1.0]  GraphicShininess=75  DoExposeReferenceFrame=on  SerializedFrames=<Frames/>
  ring_B : sm_lib/Body Elements/File Solid  ExtGeomFileName=C:/Capstone1/models/rev5/source/meshes/ring_B.stl  UnitType=Custom  ExtGeomFileUnits=mm  StepReaderType=HEX  ExportConvexHullGeometry=off  InertiaType=Custom  BasedOnType=DensityFromFile  Density=1000  DensityUnits=kg/m^3  Mass=0.0006658605629283556  MassUnits=kg  CenterOfMass=[-0.02 -2.454131698660125e-18 0.01800000000000001]  CenterOfMassUnits=m  MomentsOfInertia=[1.365014154003102e-08 7.324466192211724e-09 7.324466192211512e-09]  MomentsOfInertiaUnits=kg*m^2  ProductsOfInertia=[1.688579831515823e-23 -5.293955920339377e-23 -2.723515857283582e-24]  ProductsOfInertiaUnits=kg*m^2  GraphicType=FromGeometry  MarkerShape=Sphere  MarkerSize=10  GraphicVisPropType=SimpleVisualProperties  GraphicDiffuseColor=[.89 .48 .19]  GraphicOpacity=1  GraphicSpecularColor=[0.5 0.5 0.5 1.0]  GraphicAmbientColor=[0.15 0.15 0.15 1.0]  GraphicEmissiveColor=[0.0 0.0 0.0 1.0]  GraphicShininess=75  DoExposeReferenceFrame=on  SerializedFrames=<Frames/>
  slipring_SZH-SLI020_PLACEHOLDER : sm_lib/Body Elements/File Solid  ExtGeomFileName=C:/Capstone1/models/rev5/source/meshes/slipring_SZH-SLI020_PLACEHOLDER.stl  UnitType=Custom  ExtGeomFileUnits=mm  StepReaderType=HEX  ExportConvexHullGeometry=off  InertiaType=Custom  BasedOnType=DensityFromFile  Density=1000  DensityUnits=kg/m^3  Mass=0.0950153429495964  MassUnits=kg  CenterOfMass=[9.32744475233623e-14 5.870378722598168e-18 -0.08632108763023062]  CenterOfMassUnits=m  MomentsOfInertia=[1.142833141516155e-05 1.142833136470701e-05 1.010765604115547e-05]  MomentsOfInertiaUnits=kg*m^2  ProductsOfInertia=[5.782961395814038e-20 6.185693900914913e-17 1.11555209514856e-20]  ProductsOfInertiaUnits=kg*m^2  GraphicType=FromGeometry  MarkerShape=Sphere  MarkerSize=10  GraphicVisPropType=SimpleVisualProperties  GraphicDiffuseColor=[.42 .43 .46]  GraphicOpacity=1  GraphicSpecularColor=[0.5 0.5 0.5 1.0]  GraphicAmbientColor=[0.15 0.15 0.15 1.0]  GraphicEmissiveColor=[0.0 0.0 0.0 1.0]  GraphicShininess=75  DoExposeReferenceFrame=on  SerializedFrames=<Frames/>
  slipring_bracket : sm_lib/Body Elements/File Solid  ExtGeomFileName=C:/Capstone1/models/rev5/source/meshes/slipring_bracket.stl  UnitType=Custom  ExtGeomFileUnits=mm  StepReaderType=HEX  ExportConvexHullGeometry=off  InertiaType=Custom  BasedOnType=DensityFromFile  Density=1000  DensityUnits=kg/m^3  Mass=0.1436747351231029  MassUnits=kg  CenterOfMass=[-0.001981940292079438 3.882213856832705e-17 -0.0985]  CenterOfMassUnits=m  MomentsOfInertia=[8.479741941885203e-05 7.446851240407973e-05 0.0001590504197202461]  MomentsOfInertiaUnits=kg*m^2  ProductsOfInertia=[-1.952216166500876e-20 -5.082197683525802e-20 1.674335469965459e-19]  ProductsOfInertiaUnits=kg*m^2  GraphicType=FromGeometry  MarkerShape=Sphere  MarkerSize=10  GraphicVisPropType=SimpleVisualProperties  GraphicDiffuseColor=[.42 .43 .46]  GraphicOpacity=1  GraphicSpecularColor=[0.5 0.5 0.5 1.0]  GraphicAmbientColor=[0.15 0.15 0.15 1.0]  GraphicEmissiveColor=[0.0 0.0 0.0 1.0]  GraphicShininess=75  DoExposeReferenceFrame=on  SerializedFrames=<Frames/>
  top_plate_Al_3t : sm_lib/Body Elements/File Solid  ExtGeomFileName=C:/Capstone1/models/rev5/source/meshes/top_plate_Al_3t.stl  UnitType=Custom  ExtGeomFileUnits=mm  StepReaderType=HEX  ExportConvexHullGeometry=off  InertiaType=Custom  BasedOnType=DensityFromFile  Density=1000  DensityUnits=kg/m^3  Mass=0.04208497467862233  MassUnits=kg  CenterOfMass=[1.00014627316237e-14 -1.00288140426491e-16 -0.001506367019684553]  CenterOfMassUnits=m  MomentsOfInertia=[3.481872907036933e-05 3.448663764666895e-05 6.924242130442234e-05]  MomentsOfInertiaUnits=kg*m^2  ProductsOfInertia=[-1.316052975449905e-21 -1.294905126206455e-19 -1.660457114888754e-07]  ProductsOfInertiaUnits=kg*m^2  GraphicType=FromGeometry  MarkerShape=Sphere  MarkerSize=10  GraphicVisPropType=SimpleVisualProperties  GraphicDiffuseColor=[.42 .43 .46]  GraphicOpacity=1  GraphicSpecularColor=[0.5 0.5 0.5 1.0]  GraphicAmbientColor=[0.15 0.15 0.15 1.0]  GraphicEmissiveColor=[0.0 0.0 0.0 1.0]  GraphicShininess=75  DoExposeReferenceFrame=on  SerializedFrames=<Frames/>
  wires:
  Angles from state/1 -> Arm angle PS/1
  Angles from state/2 -> CAD upright offset/1
  CAD upright offset/1 -> Pendulum angle PS/1
  Angles from state/3 -> Unused rates/1
  True state/1 -> Select failure replay/3
  Recorded failed state/1 -> Select failure replay/1
  Failure replay enable/1 -> Select failure replay/2
  Select failure replay/1 -> Angles from state/1, Displayed state log/1
  connections:
  Mechanism/RConn1 -- World/RConn1 -- box_lid_rev5/RConn1 -- electronics_box_rev5/RConn1 -- slipring_bracket/RConn1 -- module_DC_SSR/RConn1 -- module_terminal_block/RConn1 -- module_48V_5V_converter/RConn1 -- E-stop_22mm_placeholder/RConn1 -- SEENGREAT_RS485_Dual_CAN_HAT/RConn1 -- Raspberry_Pi_5/RConn1 -- SPCC_plate_146x146x3_2/RConn1 -- slipring_SZH-SLI020_PLACEHOLDER/RConn1 -- top_plate_Al_3t/RConn1 -- RMD-X6-P20-60-E/RConn1 -- base_link/RConn1 -- Vertical arm joint/LConn1 -- Multibody solver/RConn1
  Arm angle PS/RConn1 -- Vertical arm joint/LConn2
  Rev5 hinge frame/LConn1 -- Vertical arm joint/RConn1 -- 688ZZ_A/RConn1 -- arm_holder/RConn1 -- hub_rev5/RConn1 -- 688ZZ_B/RConn1 -- encoder_pod_rev5/RConn1 -- encoder_pod_cover_rev5/RConn1 -- Grove_AS5600_PCB/RConn1 -- Grove_connector/RConn1 -- Grove_switch/RConn1 -- AS5600_chip/RConn1 -- drive_tube_6x4/RConn1
  Rev5 hinge frame/RConn1 -- Horizontal pendulum joint/LConn1
  Pendulum angle PS/RConn1 -- Horizontal pendulum joint/LConn2
  Horizontal pendulum joint/RConn1 -- Pendulum CAD origin/LConn1
  ring_B/RConn1 -- Pendulum CAD origin/RConn1 -- magnet_insert_rev4/RConn1 -- magnet_6x3_diametric/RConn1 -- ring_A/RConn1 -- bending_pipe/RConn1

== system furuta_block_model_fixed/02 Pi - Sensor and RMD Diagnostics/RMD read requests ==
  Payload : Inport
  Enable : EnablePort
  CAN Transmit : raspberrypiCommlib/CAN Transmit  DeviceID=can0  SetupCAN=off  TypeofCAN=Real  InputDataType=Raw data  BlockingMode_=off  BlockTimeout_=1  OutputStatus=off  IdentifierType=Standard (11-bit identifier)  MessageId=321  MsgLength=8  RemoteFrame=off  SimulateUsing=Code generation
  CAN payload 8x1 : Reshape  OutputDimensionality=Customize  OutputDimensions=[8 1]
  wires:
  Payload/1 -> CAN payload 8x1/1
  CAN payload 8x1/1 -> CAN Transmit/1

== system furuta_block_model_fixed/03 Pi - Motor Control and Telemetry/Angle request 0x92 ==
  Enable : EnablePort
  CAN Transmit : raspberrypiCommlib/CAN Transmit  DeviceID=can0  SetupCAN=off  TypeofCAN=Real  InputDataType=Raw data  BlockingMode_=off  BlockTimeout_=1  OutputStatus=off  IdentifierType=Standard (11-bit identifier)  MessageId=321  MsgLength=8  RemoteFrame=off  SimulateUsing=Code generation
  CAN payload 8x1 : Reshape  OutputDimensionality=Customize  OutputDimensions=[8 1]
  Payload : Constant  Value=uint8([146 0 0 0 0 0 0 0])  SampleTime=.005
  wires:
  Payload/1 -> CAN payload 8x1/1
  CAN payload 8x1/1 -> CAN Transmit/1

== system furuta_block_model_fixed/03 Pi - Motor Control and Telemetry/Motor CAN transmit ==
  Payload : Inport
  Enable : EnablePort
  CAN Transmit : raspberrypiCommlib/CAN Transmit  DeviceID=can0  SetupCAN=off  TypeofCAN=Real  InputDataType=Raw data  BlockingMode_=off  BlockTimeout_=1  OutputStatus=off  IdentifierType=Standard (11-bit identifier)  MessageId=321  MsgLength=8  RemoteFrame=off  SimulateUsing=Code generation
  CAN payload 8x1 : Reshape  OutputDimensionality=Customize  OutputDimensions=[8 1]
  wires:
  Payload/1 -> CAN payload 8x1/1
  CAN payload 8x1/1 -> CAN Transmit/1

== system furuta_block_model_fixed/01 MIL - Controller and Plant/03 Controllers/LMPC (sim) ==
  mode : Inport
  x : Inport  Port=2
  LMPC Hessian : Constant  Value=lmpcH
  LMPC bounded QP : MATLAB Function  Commented=on  TreatAsAtomicUnit=on
  LMPC state term : Constant  Value=lmpcF
  u : Outport
  wires:
  mode/1 -> LMPC bounded QP/2(mode)
  LMPC bounded QP/1(u) -> u/1
  LMPC Hessian/1 -> LMPC bounded QP/3(H)
  LMPC state term/1 -> LMPC bounded QP/4(F)
  x/1 -> LMPC bounded QP/1(x)

== system furuta_block_model_fixed/01 MIL - Controller and Plant/03 Controllers/LQR ==
  mode : Inport
  x : Inport  Port=2
  Arm reference log : ToWorkspace  VariableName=swingLQRArmHome  SaveFormat=Timeseries  SampleTime=-1
  Capture arm reference : MATLAB Function  TreatAsAtomicUnit=on
  Capture thresholds : Constant  Value=swingLqrThresholds
  Control period : Constant  Value=controlPeriod
  Energy parameters : Constant  Value=plantCoefficients
  LQR active log : ToWorkspace  VariableName=swingLqrActive  SaveFormat=Timeseries  SampleTime=-1
  LQR minus K : Gain  Gain=-lqrGain  Multiplication=Matrix(K*u) (u vector)
  Swing-up to LQR : MATLAB Function  TreatAsAtomicUnit=on
  u : Outport
  wires:
  Control period/1 -> ?
  mode/1 -> Swing-up to LQR/3(mode), Capture arm reference/2(mode)
  x/1 -> Swing-up to LQR/1(x), Capture arm reference/1(x)
  LQR minus K/1 -> Swing-up to LQR/2(balance)
  Capture thresholds/1 -> Swing-up to LQR/4(thresholds), Capture arm reference/3(thresholds)
  Energy parameters/1 -> Swing-up to LQR/5(p)
  Swing-up to LQR/1(u) -> u/1
  Swing-up to LQR/2(balancing) -> LQR active log/1
  Capture arm reference/1(relative) -> LQR minus K/1
  Capture arm reference/3(home) -> Arm reference log/1

== system furuta_block_model_fixed/01 MIL - Controller and Plant/03 Controllers/MPC Controller ==
  mo or x : Inport
  MPC Controller : mpclib/MPC Controller  SCDEnableBlockLinearizationSpecification=on  mpcobj=furutaToolboxMpc  is_multiple=0  enable_value=0  return_u0=off  updateMPCinCallerWorkspace=on  md_inport=off  mv_inport=off  uref_inport=off  return_cost=off  return_mvseq=off  return_qpstatus=off  return_xseq=off  return_state=off  return_ovseq=off  state_inport=on  umin_inport=off  umax_inport=off  ymin_inport=off  ymax_inport=off  cc_inport=off  ywt_inport=off  uwt_inport=off  duwt_inport=off  rhoeps_inport=off  pm_inport=off  MaximumP=10  HorizonChoice=FixedHorizon  n_ts=0.01  n_p=20  n_mv=1  n_md=0  n_ud=0  n_mo=8  n_uo=0  BlockDataType=double  SampleTimeInherited=off  switch_inport=off
  MPC upright reference : Constant  Value=zeros(8,1)
  mv : Outport
  wires:
  mo or x/1 -> MPC Controller/1
  MPC Controller/1 -> mv/1
  MPC upright reference/1 -> MPC Controller/2
